simulink model "Chap4_5b"  (R2020b)
settings: Solver=VariableStepAuto  StartTime=0.0  StopTime=50  RelTol=1e-3
StopFcn:
  | Plot4_5b
libraries: simulink x2
settings Model: Creator=yiyon  LastModifiedBy=yiyon

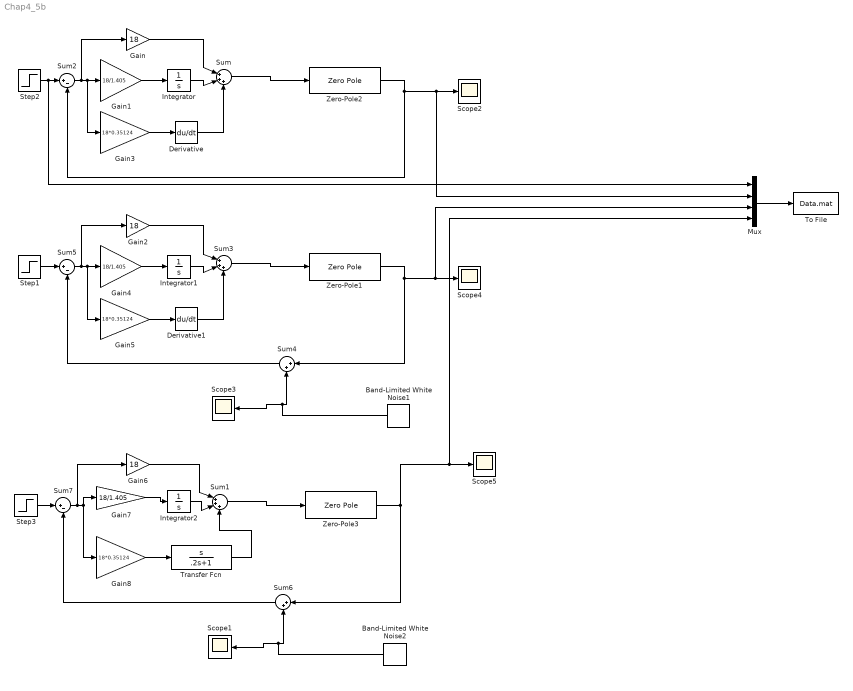
== system Chap4_5b ==
  Band-Limited White Noise1 : simulink/Sources/Band-Limited White Noise  Cov=[0.0001]  Ts=0.001  seed=[23341]
  Band-Limited White Noise2 : simulink/Sources/Band-Limited White Noise  Cov=[0.001]  Ts=0.001  seed=[23341]
  Derivative : Derivative
  Derivative1 : Derivative
  Gain : Gain  Gain=18
  Gain1 : Gain  Gain=18/1.405
  Gain2 : Gain  Gain=18
  Gain3 : Gain  Gain=18*0.35124
  Gain4 : Gain  Gain=18/1.405
  Gain5 : Gain  Gain=18*0.35124
  Gain6 : Gain  Gain=18
  Gain7 : Gain  Gain=18/1.405
  Gain8 : Gain  Gain=18*0.35124
  Integrator : Integrator
  Integrator1 : Integrator
  Integrator2 : Integrator
  Mux : Mux
  Scope{1..5} (5 alike) : Scope
  Step1 : Step  Time=0
  Step2 : Step  Time=0
  Step3 : Step  Time=0
  Sum : Sum  Inputs=|+++
  Sum1 : Sum  Inputs=|+++
  Sum2 : Sum  Inputs=|+-
  Sum3 : Sum  Inputs=|+++
  Sum4 : Sum  Inputs=|++
  Sum5 : Sum  Inputs=|+-
  Sum6 : Sum  Inputs=|++
  Sum7 : Sum  Inputs=|+-
  To File : ToFile  Filename=Data.mat  SaveFormat=Timeseries
  Transfer Fcn : TransferFcn  Numerator=[1 0]  Denominator=[.2 1]
  Zero-Pole1 : ZeroPole  Zeros=[]  Poles="[0 -1  -5]"
  Zero-Pole2 : ZeroPole  Zeros=[]  Poles="[0 -1  -5]"
  Zero-Pole3 : ZeroPole  Zeros=[]  Poles="[0 -1  -5]"
  wires:
  Step2/1 -> Mux/1, Sum2/1
  Sum/1 -> Zero-Pole2/1
  Sum2/1 -> Gain/1, Gain3/1, Gain1/1
  Gain1/1 -> Integrator/1
  Gain3/1 -> Derivative/1
  Gain/1 -> Sum/1
  Integrator/1 -> Sum/2
  Derivative/1 -> Sum/3
  Zero-Pole2/1 -> Sum2/2, Mux/2, Scope2/1
  Sum3/1 -> Zero-Pole1/1
  Sum4/1 -> Sum5/2
  Band-Limited White Noise1/1 -> Sum4/2, Scope3/1
  Derivative1/1 -> Sum3/3
  Gain4/1 -> Integrator1/1
  Sum5/1 -> Gain2/1, Gain5/1, Gain4/1
  Step1/1 -> Sum5/1
  Gain2/1 -> Sum3/1
  Gain5/1 -> Derivative1/1
  Integrator1/1 -> Sum3/2
  Zero-Pole1/1 -> Sum4/1, Mux/3, Scope4/1
  Zero-Pole3/1 -> Sum6/1, Mux/4, Scope5/1
  Integrator2/1 -> Sum1/2
  Gain8/1 -> Transfer Fcn/1
  Gain6/1 -> Sum1/1
  Gain7/1 -> Integrator2/1
  Step3/1 -> Sum7/1
  Transfer Fcn/1 -> Sum1/3
  Sum1/1 -> Zero-Pole3/1
  Sum7/1 -> Gain6/1, Gain8/1, Gain7/1
  Sum6/1 -> Sum7/2
  Band-Limited White Noise2/1 -> Sum6/2, Scope1/1
  Mux/1 -> To File/1
